simulink model "H10_JB"  (R2026a)
settings: Solver=VariableStepAuto  StopTime=2  MaxStep=2e-3
InitFcn:
  | % Modellparaméterek
  | B = 5e-4;
  | J = 500e-7;
  | 
  | % Kezdeti érték
  | omega_M0 = 100;
settings Model: Creator=Szalay  LastModifiedBy=Szalay

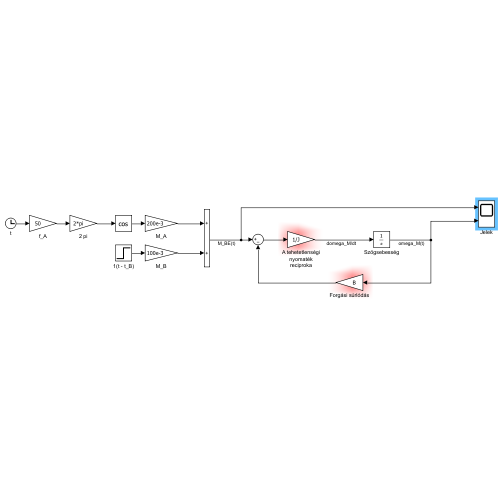
[thumbnail: Simulink's stored preview of the top-level diagram]
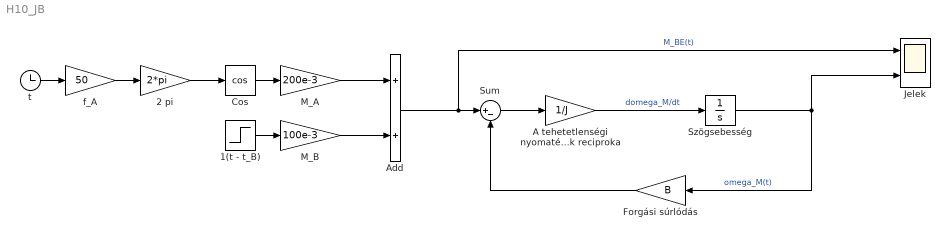
== system H10_JB ==
  1(t - t_B) : Step  Time=1250e-3  SampleTime=0
  2 pi : Gain  Gain=2*pi
  A tehetetlenségi nyomaték reciproka : Gain  Gain=1/J
  Add : Sum
  Cos : Trigonometry  Operator=cos
  Forgási súrlódás : Gain  Gain=B
  Jelek : Scope  NumInputPorts=2
      settings: ActiveDisplayYMinimum=-40.260886899598482  ActiveDisplayYMaximum=240.13151259249329
  M_A : Gain  Gain=200e-3
  M_B : Gain  Gain=100e-3
  Sum : Sum  Inputs=|+-
  Szögsebesség : Integrator  InitialCondition=omega_M0
  f_A : Gain  Gain=50
  t : Clock
  wires:
  Szögsebesség/1 -> Jelek/2, Forgási súrlódás/1  "omega_M(t)"
  A tehetetlenségi nyomaték reciproka/1 -> Szögsebesség/1  "domega_M/dt"
  Sum/1 -> A tehetetlenségi nyomaték reciproka/1
  Forgási súrlódás/1 -> Sum/2
  Add/1 -> Jelek/1, Sum/1  "M_BE(t)"
  M_A/1 -> Add/1
  Cos/1 -> M_A/1
  t/1 -> f_A/1
  f_A/1 -> 2 pi/1
  2 pi/1 -> Cos/1
  M_B/1 -> Add/2
  1(t - t_B)/1 -> M_B/1
